simulink model "SoftFinger"  (R2026b)
settings: Solver=VariableStepAuto
libraries: nesl_utility x8
settings Model: Creator=amavromm  LastModifiedBy=amavromm

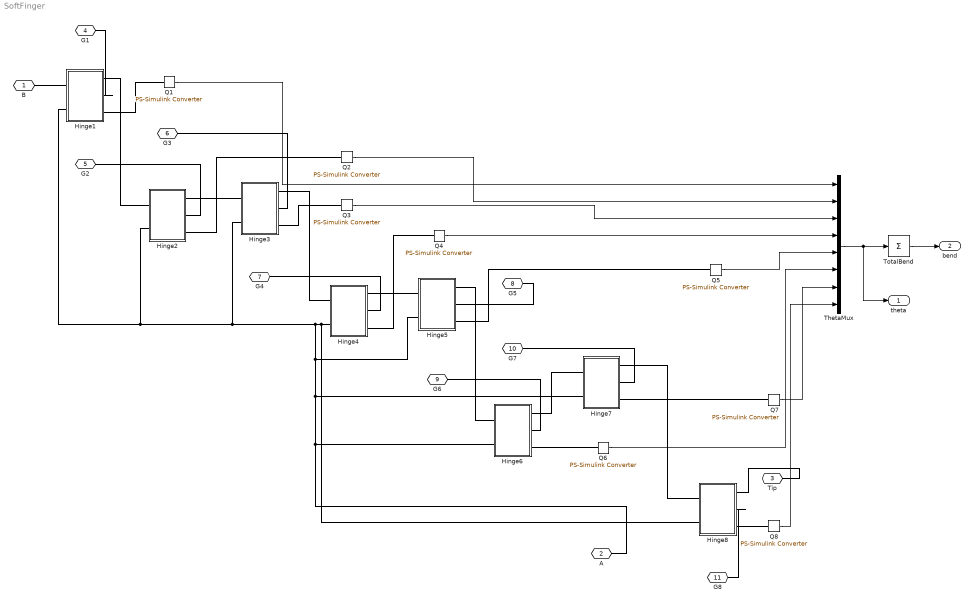
== system SoftFinger ==
  Hinge{1..8} (8 alike) : Subsystem  ReferencedSubsystem=Hinge
  Q{1..8} (8 alike) : nesl_utility/PS-Simulink Converter  PhysicalDomain=network_engine_domain  SubClassName=ps_output  LeftPortType=input  RightPortType=output  PseudoPeriodic=off  Frequencies=[]  VectorFormat=inherit  Unit=rad  AffineConversion=off
  ThetaMux : Mux  Inputs=8
  TotalBend : Sum  Inputs=+
  B : PMIOPort  Side=Left
  A : PMIOPort  Port=2  Side=Left
  Tip : PMIOPort  Port=3  Side=Right
  G1 : PMIOPort  Port=4  Side=Right
  G2 : PMIOPort  Port=5  Side=Right
  G3 : PMIOPort  Port=6  Side=Right
  G4 : PMIOPort  Port=7  Side=Right
  G5 : PMIOPort  Port=8  Side=Right
  G6 : PMIOPort  Port=9  Side=Right
  G7 : PMIOPort  Port=10  Side=Right
  G8 : PMIOPort  Port=11  Side=Right
  theta : Outport
  bend : Outport  Port=2
  wires:
  TotalBend/1 -> bend/1
  ThetaMux/1 -> theta/1, TotalBend/1
  Q8/1 -> ThetaMux/8
  Q7/1 -> ThetaMux/7
  Q6/1 -> ThetaMux/6
  Q5/1 -> ThetaMux/5
  Q4/1 -> ThetaMux/4
  Q3/1 -> ThetaMux/3
  Q2/1 -> ThetaMux/2
  Q1/1 -> ThetaMux/1
  connections:
  Hinge8/RConn3 -- Q8/LConn1
  Hinge7/RConn3 -- Q7/LConn1
  Hinge6/RConn3 -- Q6/LConn1
  Hinge5/RConn3 -- Q5/LConn1
  Hinge4/RConn3 -- Q4/LConn1
  Hinge3/RConn3 -- Q3/LConn1
  Hinge2/RConn3 -- Q2/LConn1
  Hinge1/RConn3 -- Q1/LConn1
  Hinge7/LConn2 -- Hinge6/LConn2 -- A/RConn1 -- Hinge1/LConn2 -- Hinge2/LConn2 -- Hinge3/LConn2 -- Hinge8/LConn2 -- Hinge4/LConn2 -- Hinge5/LConn2
  Hinge8/RConn2 -- G8/RConn1
  Hinge7/RConn2 -- G7/RConn1
  Hinge6/RConn2 -- G6/RConn1
  Hinge5/RConn2 -- G5/RConn1
  Hinge4/RConn2 -- G4/RConn1
  Hinge3/RConn2 -- G3/RConn1
  Hinge2/RConn2 -- G2/RConn1
  Hinge1/RConn2 -- G1/RConn1
  Hinge8/RConn1 -- Tip/RConn1
  Hinge7/RConn1 -- Hinge8/LConn1
  Hinge6/RConn1 -- Hinge7/LConn1
  Hinge5/RConn1 -- Hinge6/LConn1
  Hinge4/RConn1 -- Hinge5/LConn1
  Hinge3/RConn1 -- Hinge4/LConn1
  Hinge2/RConn1 -- Hinge3/LConn1
  Hinge1/RConn1 -- Hinge2/LConn1
  B/RConn1 -- Hinge1/LConn1
